simulink model "meteorprocess_model2"  (R2022b)
settings: Solver=VariableStepAuto  StartTime=0.0  StopTime=30.0  RelTol=1e-3
libraries: dsparch4 x2, dspvision x1
settings Model: Creator=bruce  LastModifiedBy=bruce

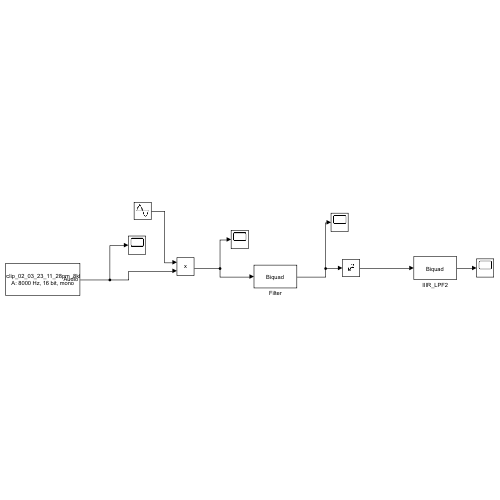
[thumbnail: Simulink's stored preview of the top-level diagram]
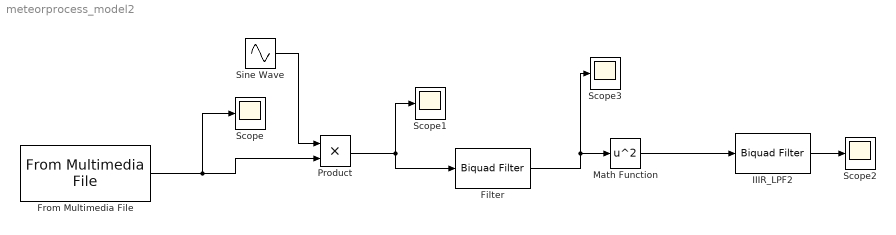
== system meteorprocess_model2 ==
  Filter : dsparch4/Biquad Filter  Tag=BlockMethodSubSystem  FilterSource=Dialog parameters  CoeffSource=Specify via dialog  FilterObject=BQF  IIRFiltStruct=Direct form II  BiQuadCoeffs=[1 2 1 1 -1.99426723116395088 0.994322417084557375;1 2 1 1 -1.98629294553082003 0.98634791078476447]  ScaleValues=[1.37964801516751179e-05;1.37413134860738063e-05;1]  IC=0  ICnum=0  ICden=0  a0Flag=Warning  optimizeScaleValues=on  ScaleValueMode=Specify via input port (g)  InputProcessing=Columns as channels (frame based)  roundingMode=Floor  overflowMode=off  scaleValueFracLength=14  denProdOutputFracLength=30  denAccumFracLength=30  secondMemoryFracLength=15
  From Multimedia File : dspvision/From Multimedia File  inputFilename=C:\Users\bruce\OneDrive\Documents\MATLAB\meteoraudio\meteorclip_02_03_23_11_28pm_8khz.wav  readRange=[1 Inf]  loop=on  numPlays=inf  outputStreams=Audio only  videoDataType=single  audioDataType=double  inheritSampleTime=on  userDefinedSampleTime=1/30  noAudioOutput=off  isIntensityVideo=off  fourcc=RGB  colorVideoFormat=Separate color signals  outputEOF=off  dataOrg=Column-major  audioFrameSize=1  computeAudioFrameSize=off  outSamplingMode=Sample based
      settings: LibrarySourceBlock=audiosources/From Multimedia File
  IIIR_LPF2 : dsparch4/Biquad Filter  Tag=BlockMethodSubSystem  FilterSource=Dialog parameters  CoeffSource=Specify via dialog  FilterObject=BQF  IIRFiltStruct=Direct form II  BiQuadCoeffs=[1 2 1 1 -1.99606514139455959 0.996126349841962799;1 1 0 1 -0.996126290566027972 0]  ScaleValues=[1.53021118508895836e-05;0.00193685471698609008;1]  IC=0  ICnum=0  ICden=0  a0Flag=Warning  optimizeScaleValues=on  ScaleValueMode=Specify via input port (g)  InputProcessing=Columns as channels (frame based)  roundingMode=Floor  overflowMode=off  scaleValueFracLength=14  denProdOutputFracLength=30  denAccumFracLength=30  secondMemoryFracLength=15
  Math Function : Math  Operator=square
  Product : Product
  Scope{,1..3} (4 alike) : Scope
  Sine Wave : Sin  Frequency=6200  SampleTime=0
  wires:
  From Multimedia File/1 -> Scope/1, Product/2
  Sine Wave/1 -> Product/1
  Product/1 -> Filter/1, Scope1/1
  Filter/1 -> Scope3/1, Math Function/1
  Math Function/1 -> IIIR_LPF2/1
  IIIR_LPF2/1 -> Scope2/1
